simulink model "ml"  (R2023b)
settings: Solver=VariableStepAuto  StartTime=0.0  StopTime=10.0  RelTol=1e-3
settings Model: Creator=Иван  LastModifiedBy=ansyser

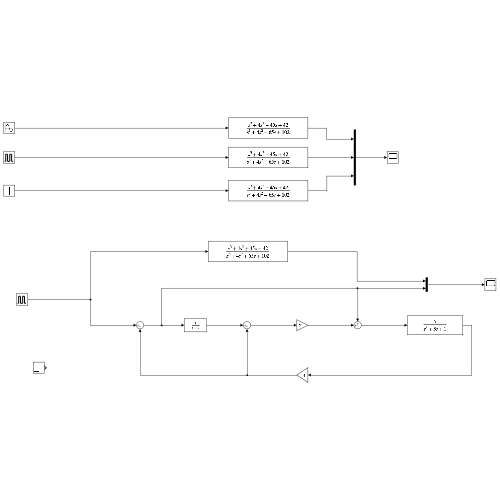
[thumbnail: Simulink's stored preview of the top-level diagram]
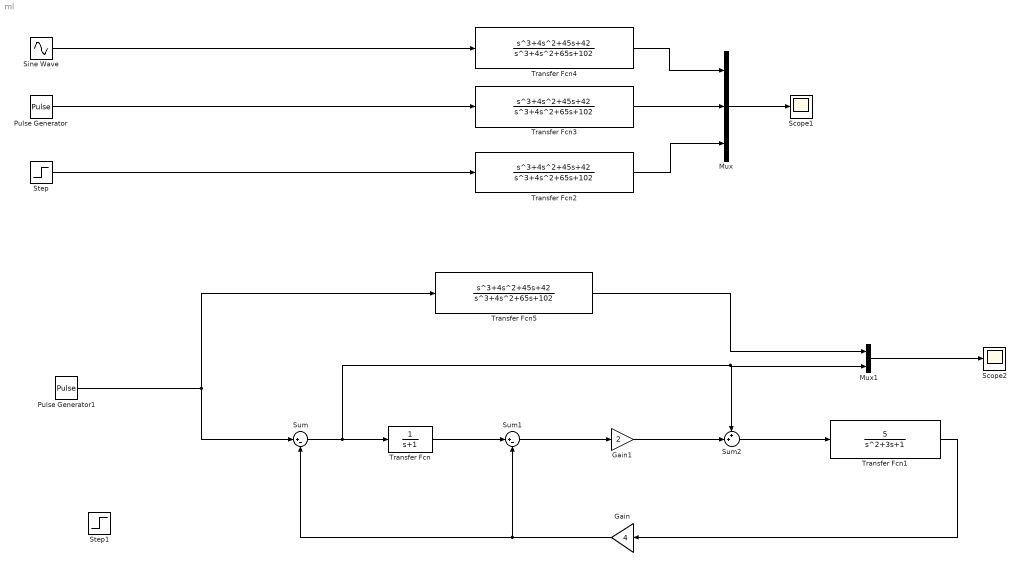
== system ml ==
  Gain : Gain  Gain=4
  Gain1 : Gain  Gain=2
  Mux : Mux  Inputs=3
  Mux1 : Mux  Inputs=2
  Pulse Generator : DiscretePulseGenerator  PulseType=Time based  Period=10  PulseWidth=5
  Pulse Generator1 : DiscretePulseGenerator  PulseType=Time based  Period=10  PulseWidth=5
  Scope1 : Scope
  Scope2 : Scope
  Sine Wave : Sin  SampleTime=0
  Step : Step  SampleTime=0
  Step1 : Step  SampleTime=0
  Sum : Sum  Inputs=|+-
  Sum1 : Sum  Inputs=|+-
  Sum2 : Sum  Inputs=++|
  Transfer Fcn : TransferFcn  Denominator=[1 1]
  Transfer Fcn1 : TransferFcn  Numerator=[5]  Denominator=[1 3 1]
  Transfer Fcn{2..5} (4 alike) : TransferFcn  Numerator=[1 4 45 42]  Denominator=[1 4 65 102]
  wires:
  Gain/1 -> Sum1/2, Sum/2
  Transfer Fcn/1 -> Sum1/1
  Sum1/1 -> Gain1/1
  Gain1/1 -> Sum2/2
  Sum2/1 -> Transfer Fcn1/1
  Transfer Fcn1/1 -> Gain/1
  Sum/1 -> Mux1/2, Sum2/1, Transfer Fcn/1
  Step/1 -> Transfer Fcn2/1
  Transfer Fcn2/1 -> Mux/3
  Pulse Generator/1 -> Transfer Fcn3/1
  Sine Wave/1 -> Transfer Fcn4/1
  Transfer Fcn3/1 -> Mux/2
  Transfer Fcn4/1 -> Mux/1
  Mux/1 -> Scope1/1
  Mux1/1 -> Scope2/1
  Pulse Generator1/1 -> Sum/1, Transfer Fcn5/1
  Transfer Fcn5/1 -> Mux1/1
